simulink model "furuta_block_model"  (R2026b)
settings: Solver=FixedStepDiscrete  StopTime=5  FixedStep=controlPeriod
model workspace (MAT data in the model file):
  controlPeriod = 0.01
  initialState = [0; 0.174532925199; 0; 0]
  integrationStep = 0.002
  lqrGain = [-0.560244322113 -7.30813603654 -0.304541725168 -0.68699829167]
  maxTorque = 0.03
  plantCoefficients = [0.00019818 0.00016078 0.00016134 0.00013805 0.016934 0.0001 1e-05 0]
  scenarioStimulus = [0 0.0075 0.0175 0.0275 0.0375 0.0475 0.0575 0.0675 0.0775 0.0875 0.0975 0.1075 ... (2004 elements, 501x4)]
  usePolicyCallback = 0
values from neighbouring files (symbols this model uses):
  C = [B A*B A^2*B A^3*B]    [build_furuta_rmd.m]
  N = 20    [build_furuta_rl.m]    (also in design_classical.m)
  pidGains = getVariable(mw,'pidGains')    [check_furuta_lqr_capture.m]
  rmd = struct('model','RMD-X6-P20-60-E','voltage',48,'gearRatio',19.612,          'ratedTorque',20,'ratedCurrent',9.5,'ratedSpeedRPM',153,          'noLoadSpeedRPM',176,'Kt',2.1,'currentLSB',.01)    [build_furuta_rmd.m]
  s = load(matFile,'ds')    [analyze_pi_current_run.m]    (also in analyze_pi_speed_run.m; build_furuta_rl.m = sin(x(2));"; build_furuta_simulink.m = s(1); design_classical.m = furuta_scenarios)
  source = [step '/1']    [add_furuta_plant_blocks.m]    (also in build_furuta_pi.m = get_param(line,'SrcPortHandle'); build_furuta_pi_hardware.m = 'Drive interlocks/3'; compare_furuta_actuators.m = get_param([harness '/Requested torque'],'PortHandles'))
  Z = expm([A B; zeros(1,5)]*p.Ts)    [furuta_linearize.m]
undefined symbols (not defined in the file or in its folder): driveElectrical, lmpcF, lmpcH, poleGain, rlRewardLevel, rmdCommandDelaySamples, sgn, useRmd, X, Y
libraries: sm_lib x36, nesl_utility x8, fl_lib x7, rllib x2, mpclib x1, slpidlib x1, ee_lib x1
(part 4 of 4)

== matlab function furuta_block_model/03 Controllers/PPO/RL observation reward termination ==
  data: x input; obs output; lastAction input; level input; mode input; reward output; done output
function [obs,reward,done] = observe(x,lastAction,level,mode)
% 상태는 현재 샘플, 보상에 쓰는 행동은 이전 샘플이다.
c = cos(x(2)); s = sin(x(2));
obs = [c;s;x(1);x(3);x(4)];
reward = c-0.01*lastAction^2;
if level == 2
    reward = reward-.001*x(4)^2-.00002*x(3)^2+double(abs(atan2(s,c))<.35);
end
done = mode == 5 && abs(x(1))>2*pi;
if done
    reward = -50;
end
end
